simulink model "TESTLat"  (R2021b)
settings: Solver=VariableStepAuto  StartTime=0.0  StopTime=10.0  RelTol=1e-3
libraries: simulink_extras x4, LPVBlockLibrary x2
settings Model: Creator=jihoo  LastModifiedBy=jihoo

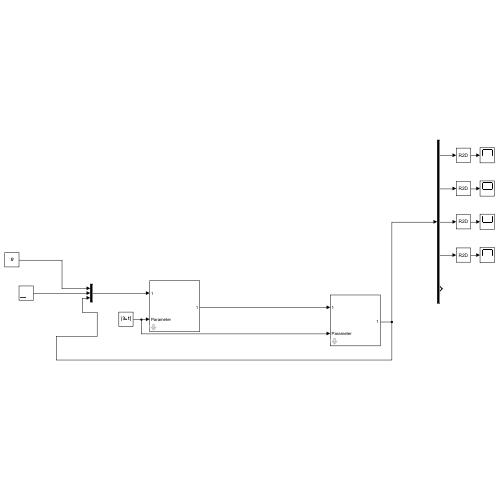
[thumbnail: Simulink's stored preview of the top-level diagram]
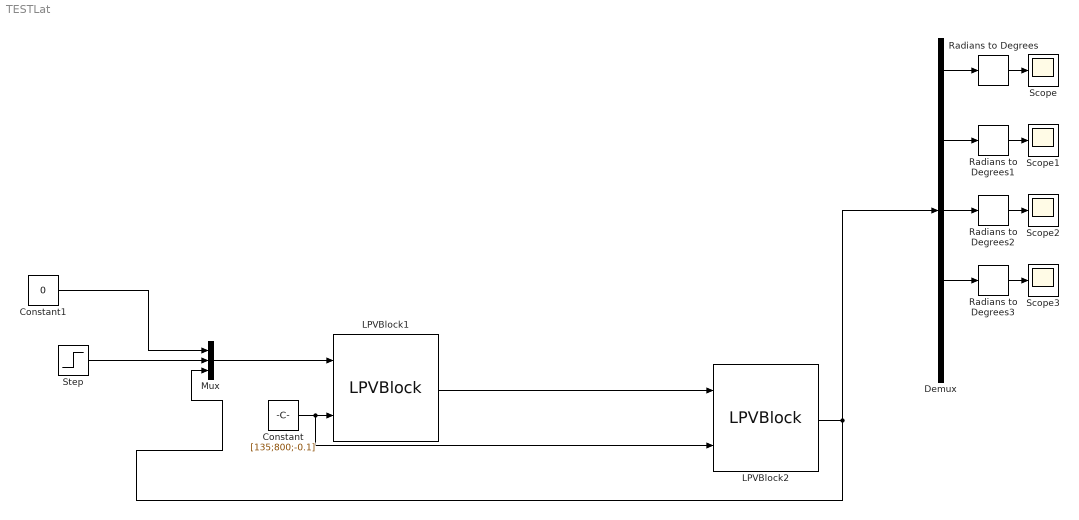
== system TESTLat ==
  Constant : Constant  Value=[135;800;-0.1]
  Constant1 : Constant  Value=0
  Demux : Demux  Outputs=5
  LPVBlock1 : LPVBlockLibrary/LPVBlock  sys=K_lat_hinf  plist={'rho1_tas_param';'rho2_alt_param';'rho3_mor_param'}  x0=0
      settings: SourceProductName=LPVTools Blocks
  LPVBlock2 : LPVBlockLibrary/LPVBlock  sys=P_lat  plist={'rho1_tas_param';'rho2_alt_param';'rho3_mor_param'}  x0=0
      settings: SourceProductName=LPVTools Blocks
  Mux : Mux  Inputs=3
  Radians to Degrees{,1..3} (4 alike) : simulink_extras/Transformations/Radians to Degrees
  Scope{,1..3} (4 alike) : Scope
  Step : Step  After=1*pi/180  SampleTime=0
  wires:
  Constant/1 -> LPVBlock2/2, LPVBlock1/2
  Mux/1 -> LPVBlock1/1
  LPVBlock1/1 -> LPVBlock2/1
  Radians to Degrees/1 -> Scope/1
  Demux/1 -> Radians to Degrees/1
  Demux/2 -> Radians to Degrees1/1
  Radians to Degrees1/1 -> Scope1/1
  Radians to Degrees2/1 -> Scope2/1
  Radians to Degrees3/1 -> Scope3/1
  Demux/4 -> Radians to Degrees3/1
  Demux/3 -> Radians to Degrees2/1
  Step/1 -> Mux/2
  LPVBlock2/1 -> Mux/3, Demux/1
  Constant1/1 -> Mux/1
